simulink model "fft_biplex_test"  (Simulink 7.4)
settings: Solver=VariableStepDiscrete  StartTime=0.0  StopTime=2000  RelTol=1e-3
libraries: xbsIndex_r4 x808, casper_library_misc x46, casper_library_delays x10, casper_library_reorder x2, casper_library_ffts_twiddle x1
(part 3 of 8)

== system fft_biplex_test/fft_biplex/biplex_core/fft_stage_7 ==
  in1 : Inport  OutDataType=sfix(16)  OutScaling=2^0
  in2 : Inport  Port=2  OutDataType=sfix(16)  OutScaling=2^0
  of_in : Inport  Port=3  OutDataType=sfix(16)  OutScaling=2^0
  sync : Inport  Port=4  OutDataType=sfix(16)  OutScaling=2^0
  shift : Inport  Port=5  OutDataType=sfix(16)  OutScaling=2^0
  Counter : xbsIndex_r4/Counter  cnt_type=Free Running  cnt_to=Inf  operation=Up  start_count=0  cnt_by_val=1  arith_type=Unsigned  n_bits=FFTSize-FFTStage+1  bin_pt=0  load_pin=off  rst=on  en=off  explicit_period=off  period=1  dbl_ovrd=off  use_behavioral_HDL=off  implementation=Fabric  use_rpm=off  block_type=counter
      settings: xl_area=[0, 0, 0, 0, 0, 0, 0]  block_version=9.1.01
  Delay : xbsIndex_r4/Delay  en=off  latency=1  dbl_ovrd=off  reg_retiming=off  block_type=delay
      settings: xl_area=[0, 0, 0, 0, 0, 0, 0]  block_version=9.1.01
  Logical1 : xbsIndex_r4/Logical  logical_function=OR  inputs=2  en=off  latency=1  precision=Full  arith_type=Unsigned  n_bits=8  bin_pt=2  align_bp=on  dbl_ovrd=off  block_type=logical
      settings: xl_area=[0, 0, 0, 0, 0, 0, 0]  block_version=9.1.01
  Mux : xbsIndex_r4/Mux  inputs=2  en=off  latency=1  precision=Full  arith_type="Signed  (2's comp)"  n_bits=8  bin_pt=2  quantization=Truncate  overflow=Wrap  dbl_ovrd=off  block_type=mux
      settings: xl_area=[0, 0, 0, 0, 0, 0, 0]  block_version=9.1.01
  Mux1 : xbsIndex_r4/Mux  inputs=2  en=off  latency=1  precision=Full  arith_type="Signed  (2's comp)"  n_bits=8  bin_pt=2  quantization=Truncate  overflow=Wrap  dbl_ovrd=off  block_type=mux
      settings: xl_area=[0, 0, 0, 0, 0, 0, 0]  block_version=9.1.01
  Slice : xbsIndex_r4/Slice  nbits=1  boolean_output=on  mode=Lower Bit Location + Width  bit1=-(FFTStage - 1)  base1=MSB of Input  bit0=FFTStage - 1  base0=LSB of Input  dbl_ovrd=off  block_type=slice
      settings: infoedit="Extracts a given range of bits from each input sample and presents it at the output.  The output type is ordinarily unsigned with binary point at zero, but can be Boolean when the slice is one bit wide.<P><P>Hardware notes: In hardware this block costs nothing."  block_version=9.1.01
  Slice1 : xbsIndex_r4/Slice  nbits=1  boolean_output=off  mode=Upper Bit Location + Width  bit1=0  base1=MSB of Input  bit0=0  base0=LSB of Input  dbl_ovrd=off  block_type=slice
      settings: infoedit="Extracts a given range of bits from each input sample and presents it at the output.  The output type is ordinarily unsigned with binary point at zero, but can be Boolean when the slice is one bit wide.<P><P>Hardware notes: In hardware this block costs nothing."  block_version=9.1.01
  butterfly_direct : Subsystem  AncestorBlock=casper_library_ffts/butterfly_direct  mask(butterfly_direct){biplex=on, FFTSize=8, Coeffs=getfield( getfield( get_param( gcb,'UserData' ), 'parameters'),'Coeffs'), StepPeriod=1, coeff_bit_width=12, input_bit_width=12, downshift=off, add_latency=2, mult_latency=3, bram_latency=2, conv_latency=2, quantization=Round  (unbiased: +/- Inf), overflow=Saturate, arch=Virtex2Pro, opt_target=multipliers, coeffs_bram=on, use_hdl=on, use_embedded=off, hardcode_shifts=off, dsp48_adders=off}
      mask prompts: biplex "Used in biplex FFT"; FFTSize "Size of FFT: (2^? pts)"; Coeffs "Coefficients: (0 to 2^(FFTSize-1)-1)"; StepPeriod "Coefficient Step Period: (2^?)"; coeff_bit_width "Coefficient Bit Width"; input_bit_width "Input/Output Bit Width:"; add_latency "Add Latency"; mult_latency "Mult Latency"; bram_latency "BRAM Latency"; conv_latency "Convert latency"; quantization "Quantization Behavior"; overflow "Overflow Behavior"; arch "Architecture"; opt_target "Use less"; coeffs_bram "Store coefficients in BRAM"; use_hdl "Use behavioural HDL for multipliers"; use_embedded "Use embedded multipliers"; hardcode_shifts "Hardcode shift schedule"; dsp48_adders "Use DSP48s for adders"
      mask help: FFT internal block.
      mask init: same as fft_biplex_test/fft_biplex/biplex_core/fft_stage_1/butterfly_direct
      settings: AttributesFormatString=|
      | twiddle_general_3mult
      | coeffs in BRAM
      mask StyleString: checkbox,edit,edit,edit,edit,edit,checkbox,edit,edit,edit,edit,popup(Truncate|Round  (unbiased: +/- Inf)|Round  (unbiased: Even Values)),popup(Wrap|Saturate|Error),popup(Virtex2Pro|Virtex5),popup(logic|multipliers),checkbox,checkbox,checkbox,checkbox,checkbox
      mask CallbackString:
      | ||Coeffs = get_param(gcb, 'Coeffs');
      | if (length(eval(Coeffs)) == 1),
      |     set_param_state(gcb, 'StepPeriod', 'off');
      |     set_param_state(gcb, 'coeffs_bram', 'off');
      |     set_param_state(gcb, 'coeff_bit_width', 'off');
      | else
      |     set_param_state(gcb, 'StepPeriod', 'on');
      |     set_param_state(gcb, 'coeffs_bram', 'on');
      |     set_param_state(gcb, 'coeff_bit_width', 'on');
      | end|||||||||||fft_callback_arch(gcb);|||% make mutually exclusive with use_embedded.
      | 
      | use_hdl = get_param(gcb, 'use_hdl');
      | if strcmp(use_hdl, 'on'),
      |     set_param_state(gcb, 'use_embedded', 'off');
      | else
      |     set_param_state(gcb, 'use_embedded', 'on');
      | end|% make mutually exclusive with use_hdl.
      | 
      | use_hdl = get_param(gcb, 'use_embedded');
      | if strcmp(use_hdl, 'on'),
      |     set_param_state(gcb, 'use_hdl', 'off');
      | else
      |     set_param_state(gcb, 'use_hdl', 'on');
      | end|hardcode_shifts = get_param(gcb, 'hardcode_shifts');
      | set_param_state(gcb, 'downshift', hardcode_shifts);|fft_callback_dsp48_adders(gcb);
      mask TabNameString: Basic,Basic,Basic,Basic,Basic,Basic,Basic,Latency,Latency,Latency,Latency,Implementation,Implementation,Implementation,Implementation,Implementation,Implementation,Implementation,Implementation,Implementation
  delay_b : Subsystem  AncestorBlock=casper_library_delays/delay_slr  mask(delay_slr){DelayLen=2^(FFTSize-FFTStage)}
      mask prompts: DelayLen "Delay by:"
      mask help: A delay block that uses slices (SLR16s) for its storage.
      mask Help: eval('xlWeb(''http://casper.berkeley.edu/wiki/Delay_slr'')')
  delay_f : Subsystem  AncestorBlock=casper_library_delays/delay_slr  mask(delay_slr){DelayLen=2^(FFTSize-FFTStage)}
      mask prompts: DelayLen "Delay by:"
      mask help: A delay block that uses slices (SLR16s) for its storage.
      mask Help: eval('xlWeb(''http://casper.berkeley.edu/wiki/Delay_slr'')')
  sync_delay : casper_library_delays/sync_delay  SystemSampleTime=-1  DelayLen=2^(FFTSize - FFTStage)
  out1 : Outport  OutDataType=sfix(16)  OutScaling=2^0
  out2 : Outport  Port=2  OutDataType=sfix(16)  OutScaling=2^0
  of : Outport  Port=3  OutDataType=sfix(16)  OutScaling=2^0
  sync_out : Outport  Port=4  OutDataType=sfix(16)  OutScaling=2^0
  wires:
  shift/1 -> Slice/1
  of_in/1 -> Logical1/2
  Logical1/1 -> of/1
  Delay/1 -> sync_delay/1
  sync/1 -> Counter/1, Delay/1
  Counter/1 -> Slice1/1
  Mux/1 -> butterfly_direct/2(b)
  Mux1/1 -> delay_b/1(In1)
  delay_f/1(Out1) -> Mux1/3, Mux/2
  in1/1 -> Mux/3, Mux1/2
  Slice1/1 -> Mux/1, Mux1/1
  in2/1 -> delay_f/1(In1)
  delay_b/1(Out1) -> butterfly_direct/1(a)
  sync_delay/1 -> butterfly_direct/3(sync)
  Slice/1 -> butterfly_direct/4(shift)
  butterfly_direct/1(a+bw) -> out1/1
  butterfly_direct/2(a-bw) -> out2/1
  butterfly_direct/3(of) -> Logical1/1
  butterfly_direct/4(sync_out) -> sync_out/1

== system fft_biplex_test/fft_biplex/biplex_core/fft_stage_8 ==
  in1 : Inport  OutDataType=sfix(16)  OutScaling=2^0
  in2 : Inport  Port=2  OutDataType=sfix(16)  OutScaling=2^0
  of_in : Inport  Port=3  OutDataType=sfix(16)  OutScaling=2^0
  sync : Inport  Port=4  OutDataType=sfix(16)  OutScaling=2^0
  shift : Inport  Port=5  OutDataType=sfix(16)  OutScaling=2^0
  Counter : xbsIndex_r4/Counter  cnt_type=Free Running  cnt_to=Inf  operation=Up  start_count=0  cnt_by_val=1  arith_type=Unsigned  n_bits=FFTSize-FFTStage+1  bin_pt=0  load_pin=off  rst=on  en=off  explicit_period=off  period=1  dbl_ovrd=off  use_behavioral_HDL=off  implementation=Fabric  use_rpm=off  block_type=counter
      settings: xl_area=[0, 0, 0, 0, 0, 0, 0]  block_version=9.1.01
  Delay : xbsIndex_r4/Delay  en=off  latency=1  dbl_ovrd=off  reg_retiming=off  block_type=delay
      settings: xl_area=[0, 0, 0, 0, 0, 0, 0]  block_version=9.1.01
  Logical1 : xbsIndex_r4/Logical  logical_function=OR  inputs=2  en=off  latency=1  precision=Full  arith_type=Unsigned  n_bits=8  bin_pt=2  align_bp=on  dbl_ovrd=off  block_type=logical
      settings: xl_area=[0, 0, 0, 0, 0, 0, 0]  block_version=9.1.01
  Mux : xbsIndex_r4/Mux  inputs=2  en=off  latency=1  precision=Full  arith_type="Signed  (2's comp)"  n_bits=8  bin_pt=2  quantization=Truncate  overflow=Wrap  dbl_ovrd=off  block_type=mux
      settings: xl_area=[0, 0, 0, 0, 0, 0, 0]  block_version=9.1.01
  Mux1 : xbsIndex_r4/Mux  inputs=2  en=off  latency=1  precision=Full  arith_type="Signed  (2's comp)"  n_bits=8  bin_pt=2  quantization=Truncate  overflow=Wrap  dbl_ovrd=off  block_type=mux
      settings: xl_area=[0, 0, 0, 0, 0, 0, 0]  block_version=9.1.01
  Slice : xbsIndex_r4/Slice  nbits=1  boolean_output=on  mode=Lower Bit Location + Width  bit1=-(FFTStage - 1)  base1=MSB of Input  bit0=FFTStage - 1  base0=LSB of Input  dbl_ovrd=off  block_type=slice
      settings: infoedit="Extracts a given range of bits from each input sample and presents it at the output.  The output type is ordinarily unsigned with binary point at zero, but can be Boolean when the slice is one bit wide.<P><P>Hardware notes: In hardware this block costs nothing."  block_version=9.1.01
  Slice1 : xbsIndex_r4/Slice  nbits=1  boolean_output=off  mode=Upper Bit Location + Width  bit1=0  base1=MSB of Input  bit0=0  base0=LSB of Input  dbl_ovrd=off  block_type=slice
      settings: infoedit="Extracts a given range of bits from each input sample and presents it at the output.  The output type is ordinarily unsigned with binary point at zero, but can be Boolean when the slice is one bit wide.<P><P>Hardware notes: In hardware this block costs nothing."  block_version=9.1.01
  butterfly_direct : Subsystem  AncestorBlock=casper_library_ffts/butterfly_direct  mask(butterfly_direct){biplex=on, FFTSize=8, Coeffs=getfield( getfield( get_param( gcb,'UserData' ), 'parameters'),'Coeffs'), StepPeriod=0, coeff_bit_width=12, input_bit_width=12, downshift=off, add_latency=2, mult_latency=3, bram_latency=2, conv_latency=2, quantization=Round  (unbiased: +/- Inf), overflow=Saturate, arch=Virtex2Pro, opt_target=multipliers, coeffs_bram=on, use_hdl=on, use_embedded=off, hardcode_shifts=off, dsp48_adders=off}
      mask prompts: biplex "Used in biplex FFT"; FFTSize "Size of FFT: (2^? pts)"; Coeffs "Coefficients: (0 to 2^(FFTSize-1)-1)"; StepPeriod "Coefficient Step Period: (2^?)"; coeff_bit_width "Coefficient Bit Width"; input_bit_width "Input/Output Bit Width:"; add_latency "Add Latency"; mult_latency "Mult Latency"; bram_latency "BRAM Latency"; conv_latency "Convert latency"; quantization "Quantization Behavior"; overflow "Overflow Behavior"; arch "Architecture"; opt_target "Use less"; coeffs_bram "Store coefficients in BRAM"; use_hdl "Use behavioural HDL for multipliers"; use_embedded "Use embedded multipliers"; hardcode_shifts "Hardcode shift schedule"; dsp48_adders "Use DSP48s for adders"
      mask help: FFT internal block.
      mask init: same as fft_biplex_test/fft_biplex/biplex_core/fft_stage_1/butterfly_direct
      settings: AttributesFormatString=|
      | twiddle_general_3mult
      | coeffs in BRAM
      mask StyleString: checkbox,edit,edit,edit,edit,edit,checkbox,edit,edit,edit,edit,popup(Truncate|Round  (unbiased: +/- Inf)|Round  (unbiased: Even Values)),popup(Wrap|Saturate|Error),popup(Virtex2Pro|Virtex5),popup(logic|multipliers),checkbox,checkbox,checkbox,checkbox,checkbox
      mask CallbackString:
      | ||Coeffs = get_param(gcb, 'Coeffs');
      | if (length(eval(Coeffs)) == 1),
      |     set_param_state(gcb, 'StepPeriod', 'off');
      |     set_param_state(gcb, 'coeffs_bram', 'off');
      |     set_param_state(gcb, 'coeff_bit_width', 'off');
      | else
      |     set_param_state(gcb, 'StepPeriod', 'on');
      |     set_param_state(gcb, 'coeffs_bram', 'on');
      |     set_param_state(gcb, 'coeff_bit_width', 'on');
      | end|||||||||||fft_callback_arch(gcb);|||% make mutually exclusive with use_embedded.
      | 
      | use_hdl = get_param(gcb, 'use_hdl');
      | if strcmp(use_hdl, 'on'),
      |     set_param_state(gcb, 'use_embedded', 'off');
      | else
      |     set_param_state(gcb, 'use_embedded', 'on');
      | end|% make mutually exclusive with use_hdl.
      | 
      | use_hdl = get_param(gcb, 'use_embedded');
      | if strcmp(use_hdl, 'on'),
      |     set_param_state(gcb, 'use_hdl', 'off');
      | else
      |     set_param_state(gcb, 'use_hdl', 'on');
      | end|hardcode_shifts = get_param(gcb, 'hardcode_shifts');
      | set_param_state(gcb, 'downshift', hardcode_shifts);|fft_callback_dsp48_adders(gcb);
      mask TabNameString: Basic,Basic,Basic,Basic,Basic,Basic,Basic,Latency,Latency,Latency,Latency,Implementation,Implementation,Implementation,Implementation,Implementation,Implementation,Implementation,Implementation,Implementation
  delay_b : Subsystem  AncestorBlock=casper_library_delays/delay_slr  mask(delay_slr){DelayLen=2^(FFTSize-FFTStage)}
      mask prompts: DelayLen "Delay by:"
      mask help: A delay block that uses slices (SLR16s) for its storage.
      mask Help: eval('xlWeb(''http://casper.berkeley.edu/wiki/Delay_slr'')')
  delay_f : Subsystem  AncestorBlock=casper_library_delays/delay_slr  mask(delay_slr){DelayLen=2^(FFTSize-FFTStage)}
      mask prompts: DelayLen "Delay by:"
      mask help: A delay block that uses slices (SLR16s) for its storage.
      mask Help: eval('xlWeb(''http://casper.berkeley.edu/wiki/Delay_slr'')')
  sync_delay : casper_library_delays/sync_delay  SystemSampleTime=-1  DelayLen=2^(FFTSize - FFTStage)
  out1 : Outport  OutDataType=sfix(16)  OutScaling=2^0
  out2 : Outport  Port=2  OutDataType=sfix(16)  OutScaling=2^0
  of : Outport  Port=3  OutDataType=sfix(16)  OutScaling=2^0
  sync_out : Outport  Port=4  OutDataType=sfix(16)  OutScaling=2^0
  wires:
  shift/1 -> Slice/1
  of_in/1 -> Logical1/2
  Logical1/1 -> of/1
  Delay/1 -> sync_delay/1
  sync/1 -> Counter/1, Delay/1
  Counter/1 -> Slice1/1
  Mux/1 -> butterfly_direct/2(b)
  Mux1/1 -> delay_b/1(In1)
  delay_f/1(Out1) -> Mux1/3, Mux/2
  in1/1 -> Mux/3, Mux1/2
  Slice1/1 -> Mux/1, Mux1/1
  in2/1 -> delay_f/1(In1)
  delay_b/1(Out1) -> butterfly_direct/1(a)
  sync_delay/1 -> butterfly_direct/3(sync)
  Slice/1 -> butterfly_direct/4(shift)
  butterfly_direct/1(a+bw) -> out1/1
  butterfly_direct/2(a-bw) -> out2/1
  butterfly_direct/3(of) -> Logical1/1
  butterfly_direct/4(sync_out) -> sync_out/1

== system fft_biplex_test/fft_biplex/biplex_cplx_unscrambler/reorder ==
  sync : Inport  OutDataType=sfix(16)  OutScaling=2^0
  en : Inport  Port=2  OutDataType=sfix(16)  OutScaling=2^0
  din0 : Inport  Port=3  OutDataType=sfix(16)  OutScaling=2^0
  Counter : xbsIndex_r4/Counter  cnt_type=Count Limited  cnt_to=511  operation=Up  start_count=0  cnt_by_val=1  arith_type=Unsigned  n_bits=9  bin_pt=0  load_pin=off  rst=on  en=on  explicit_period=on  period=1  dbl_ovrd=off  use_behavioral_HDL=off  implementation=Fabric  block_type=counter
      settings: block_version=11.4
  Mux : xbsIndex_r4/Mux  inputs=2  en=off  latency=1  precision=Full  arith_type=Unsigned  n_bits=16  bin_pt=14  quantization=Truncate  overflow=Wrap  dbl_ovrd=off  block_type=mux
      settings: block_version=11.4
  Slice1 : xbsIndex_r4/Slice  nbits=1  boolean_output=off  mode=Upper Bit Location + Width  bit1=0  base1=MSB of Input  bit0=0  base0=LSB of Input  dbl_ovrd=off  block_type=slice
  Slice2 : xbsIndex_r4/Slice  nbits=8  boolean_output=off  mode=Lower Bit Location + Width  bit1=0  base1=MSB of Input  bit0=0  base0=LSB of Input  dbl_ovrd=off  block_type=slice
  bram0 : xbsIndex_r4/Single Port RAM  depth=256  initVector=sin(pi*(0:15)/16)  distributed_mem=Block RAM  write_mode=Read Before Write  rst=off  init_reg=0  en=off  latency=2  dbl_ovrd=off  optimize=Area  use_rpm=on  block_type=spram
  delay_d0 : xbsIndex_r4/Delay  en=off  latency=0  dbl_ovrd=off  reg_retiming=off  block_type=delay
      settings: block_version=11.4
  delay_din0 : xbsIndex_r4/Delay  en=off  latency=1  dbl_ovrd=off  reg_retiming=off  block_type=delay
      settings: xl_area=[0, 0, 0, 0, 0, 0, 0]  block_version=9.1.01
  delay_map1 : xbsIndex_r4/Delay  en=off  latency=0*map_latency  dbl_ovrd=off  reg_retiming=off  block_type=delay
      settings: block_version=11.4
  delay_sel : xbsIndex_r4/Delay  en=off  latency=0  dbl_ovrd=off  reg_retiming=off  block_type=delay
      settings: block_version=11.4
  delay_valid : xbsIndex_r4/Delay  en=off  latency=3  dbl_ovrd=off  reg_retiming=off  block_type=delay
      settings: xl_area=[0, 0, 0, 0, 0, 0, 0]  block_version=9.1.01
  delay_we : xbsIndex_r4/Delay  en=off  latency=0  dbl_ovrd=off  reg_retiming=off  block_type=delay
      settings: xl_area=[0, 0, 0, 0, 0, 0, 0]  block_version=9.1.01
  map1 : xbsIndex_r4/ROM  depth=256  initVector=map  distributed_mem=Distributed memory  rst=off  init_reg=0  en=off  latency=0  arith_type=Unsigned  n_bits=8  bin_pt=0  dbl_ovrd=off  optimize=Area  use_rpm=on  block_type=sprom
      settings: block_version=11.4
  post_sync_delay : xbsIndex_r4/Delay  en=off  latency=3  dbl_ovrd=off  reg_retiming=off  block_type=delay
      settings: xl_area=[0, 0, 0, 0, 0, 0, 0]  block_version=9.1.01
  pre_sync_delay : xbsIndex_r4/Delay  en=off  latency=0  dbl_ovrd=off  reg_retiming=off  block_type=delay
      settings: xl_area=[0, 0, 0, 0, 0, 0, 0]  block_version=9.1.01
  sync_delay_en : casper_library_delays/sync_delay_en  SystemSampleTime=-1  DelayLen=256
  sync_out : Outport  OutDataType=sfix(16)  OutScaling=2^0
  valid : Outport  Port=2  OutDataType=sfix(16)  OutScaling=2^0
  dout0 : Outport  Port=3  OutDataType=sfix(16)  OutScaling=2^0
  wires:
  sync/1 -> Counter/1, pre_sync_delay/1
  en/1 -> Counter/2, sync_delay_en/2, delay_we/1
  Counter/1 -> Slice1/1, Slice2/1
  Slice1/1 -> delay_sel/1
  delay_sel/1 -> Mux/1
  Slice2/1 -> delay_d0/1, map1/1
  delay_d0/1 -> Mux/2
  pre_sync_delay/1 -> sync_delay_en/1
  sync_delay_en/1 -> post_sync_delay/1
  post_sync_delay/1 -> sync_out/1
  delay_we/1 -> delay_valid/1, bram0/3
  delay_valid/1 -> valid/1
  Mux/1 -> bram0/1
  din0/1 -> delay_din0/1
  delay_din0/1 -> bram0/2
  bram0/1 -> dout0/1
  map1/1 -> delay_map1/1
  delay_map1/1 -> Mux/3

== system fft_biplex_test/fft_biplex/biplex_cplx_unscrambler/reorder1 ==
  sync : Inport  OutDataType=sfix(16)  OutScaling=2^0
  en : Inport  Port=2  OutDataType=sfix(16)  OutScaling=2^0
  din0 : Inport  Port=3  OutDataType=sfix(16)  OutScaling=2^0
  Counter : xbsIndex_r4/Counter  cnt_type=Count Limited  cnt_to=511  operation=Up  start_count=0  cnt_by_val=1  arith_type=Unsigned  n_bits=9  bin_pt=0  load_pin=off  rst=on  en=on  explicit_period=on  period=1  dbl_ovrd=off  use_behavioral_HDL=off  implementation=Fabric  block_type=counter
      settings: block_version=11.4
  Mux : xbsIndex_r4/Mux  inputs=2  en=off  latency=1  precision=Full  arith_type=Unsigned  n_bits=16  bin_pt=14  quantization=Truncate  overflow=Wrap  dbl_ovrd=off  block_type=mux
      settings: block_version=11.4
  Slice1 : xbsIndex_r4/Slice  nbits=1  boolean_output=off  mode=Upper Bit Location + Width  bit1=0  base1=MSB of Input  bit0=0  base0=LSB of Input  dbl_ovrd=off  block_type=slice
  Slice2 : xbsIndex_r4/Slice  nbits=8  boolean_output=off  mode=Lower Bit Location + Width  bit1=0  base1=MSB of Input  bit0=0  base0=LSB of Input  dbl_ovrd=off  block_type=slice
  bram0 : xbsIndex_r4/Single Port RAM  depth=256  initVector=sin(pi*(0:15)/16)  distributed_mem=Block RAM  write_mode=Read Before Write  rst=off  init_reg=0  en=off  latency=2  dbl_ovrd=off  optimize=Area  use_rpm=on  block_type=spram
  delay_d0 : xbsIndex_r4/Delay  en=off  latency=0  dbl_ovrd=off  reg_retiming=off  block_type=delay
      settings: block_version=11.4
  delay_din0 : xbsIndex_r4/Delay  en=off  latency=1  dbl_ovrd=off  reg_retiming=off  block_type=delay
      settings: xl_area=[0, 0, 0, 0, 0, 0, 0]  block_version=9.1.01
  delay_map1 : xbsIndex_r4/Delay  en=off  latency=0*map_latency  dbl_ovrd=off  reg_retiming=off  block_type=delay
      settings: block_version=11.4
  delay_sel : xbsIndex_r4/Delay  en=off  latency=0  dbl_ovrd=off  reg_retiming=off  block_type=delay
      settings: block_version=11.4
  delay_valid : xbsIndex_r4/Delay  en=off  latency=3  dbl_ovrd=off  reg_retiming=off  block_type=delay
      settings: xl_area=[0, 0, 0, 0, 0, 0, 0]  block_version=9.1.01
  delay_we : xbsIndex_r4/Delay  en=off  latency=0  dbl_ovrd=off  reg_retiming=off  block_type=delay
      settings: xl_area=[0, 0, 0, 0, 0, 0, 0]  block_version=9.1.01
  map1 : xbsIndex_r4/ROM  depth=256  initVector=map  distributed_mem=Distributed memory  rst=off  init_reg=0  en=off  latency=0  arith_type=Unsigned  n_bits=8  bin_pt=0  dbl_ovrd=off  optimize=Area  use_rpm=on  block_type=sprom
      settings: block_version=11.4
  post_sync_delay : xbsIndex_r4/Delay  en=off  latency=3  dbl_ovrd=off  reg_retiming=off  block_type=delay
      settings: xl_area=[0, 0, 0, 0, 0, 0, 0]  block_version=9.1.01
  pre_sync_delay : xbsIndex_r4/Delay  en=off  latency=0  dbl_ovrd=off  reg_retiming=off  block_type=delay
      settings: xl_area=[0, 0, 0, 0, 0, 0, 0]  block_version=9.1.01
  sync_delay_en : casper_library_delays/sync_delay_en  SystemSampleTime=-1  DelayLen=256
  sync_out : Outport  OutDataType=sfix(16)  OutScaling=2^0
  valid : Outport  Port=2  OutDataType=sfix(16)  OutScaling=2^0
  dout0 : Outport  Port=3  OutDataType=sfix(16)  OutScaling=2^0
  wires:
  sync/1 -> Counter/1, pre_sync_delay/1
  en/1 -> Counter/2, sync_delay_en/2, delay_we/1
  Counter/1 -> Slice1/1, Slice2/1
  Slice1/1 -> delay_sel/1
  delay_sel/1 -> Mux/1
  Slice2/1 -> delay_d0/1, map1/1
  delay_d0/1 -> Mux/2
  pre_sync_delay/1 -> sync_delay_en/1
  sync_delay_en/1 -> post_sync_delay/1
  post_sync_delay/1 -> sync_out/1
  delay_we/1 -> delay_valid/1, bram0/3
  delay_valid/1 -> valid/1
  Mux/1 -> bram0/1
  din0/1 -> delay_din0/1
  delay_din0/1 -> bram0/2
  bram0/1 -> dout0/1
  map1/1 -> delay_map1/1
  delay_map1/1 -> Mux/3

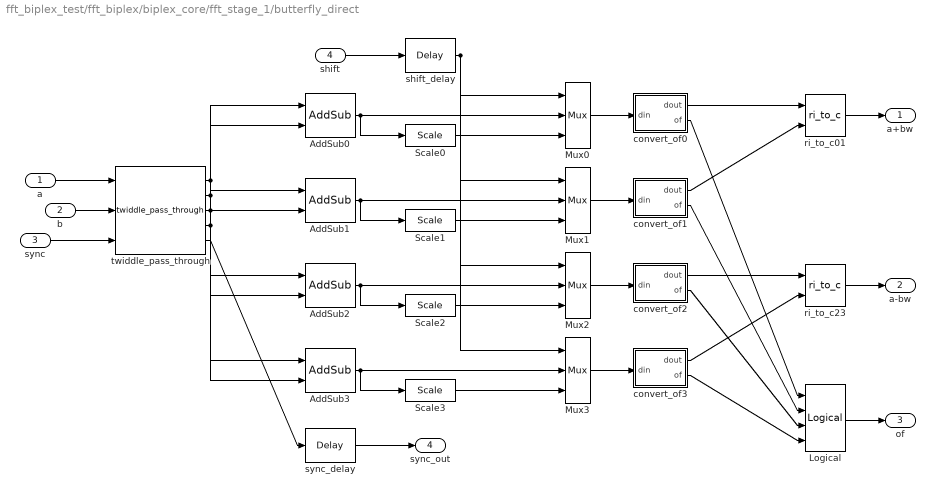
== system fft_biplex_test/fft_biplex/biplex_core/fft_stage_1/butterfly_direct ==
  a : Inport  OutDataType=sfix(16)  OutScaling=2^0
  b : Inport  Port=2  OutDataType=sfix(16)  OutScaling=2^0
  sync : Inport  Port=3  OutDataType=sfix(16)  OutScaling=2^0
  shift : Inport  Port=4  OutDataType=sfix(16)  OutScaling=2^0
  AddSub0 : xbsIndex_r4/AddSub  mode=Addition  use_carryin=off  use_carryout=off  en=off  latency=2  precision=Full  arith_type=Unsigned  n_bits=16  bin_pt=14  quantization=Truncate  overflow=Wrap  dbl_ovrd=off  use_behavioral_HDL=on  hw_selection=Fabric  pipelined=off  block_type=addsub
  AddSub1 : xbsIndex_r4/AddSub  mode=Addition  use_carryin=off  use_carryout=off  en=off  latency=2  precision=Full  arith_type=Unsigned  n_bits=16  bin_pt=14  quantization=Truncate  overflow=Wrap  dbl_ovrd=off  use_behavioral_HDL=on  hw_selection=Fabric  pipelined=off  block_type=addsub
  AddSub2 : xbsIndex_r4/AddSub  mode=Subtraction  use_carryin=off  use_carryout=off  en=off  latency=2  precision=Full  arith_type=Unsigned  n_bits=16  bin_pt=14  quantization=Truncate  overflow=Wrap  dbl_ovrd=off  use_behavioral_HDL=on  hw_selection=Fabric  pipelined=off  block_type=addsub
  AddSub3 : xbsIndex_r4/AddSub  mode=Subtraction  use_carryin=off  use_carryout=off  en=off  latency=2  precision=Full  arith_type=Unsigned  n_bits=16  bin_pt=14  quantization=Truncate  overflow=Wrap  dbl_ovrd=off  use_behavioral_HDL=on  hw_selection=Fabric  pipelined=off  block_type=addsub
  Logical : xbsIndex_r4/Logical  logical_function=OR  inputs=4  en=off  latency=0  precision=Full  arith_type=Unsigned  n_bits=16  bin_pt=0  align_bp=on  dbl_ovrd=off  block_type=logical
      settings: block_version=11.4
  Mux{0..3} (4 alike) : xbsIndex_r4/Mux  inputs=2  en=off  latency=1  precision=Full  arith_type=Unsigned  n_bits=16  bin_pt=14  quantization=Truncate  overflow=Wrap  dbl_ovrd=off  block_type=mux
      settings: block_version=11.4
  Scale{0..3} (4 alike) : xbsIndex_r4/Scale  scale_factor=-1  dbl_ovrd=off  block_type=scale
  convert_of0 : Subsystem  AncestorBlock=casper_library_misc/convert_of  mask(convert_of){bit_width_i=14, binary_point_i=12, bit_width_o=12, binary_point_o=11, latency=2, overflow=Saturate, quantization=Round  (unbiased: +/- Inf)}
      mask prompts: bit_width_i "Bit Width In"; binary_point_i "Binary Point In"; bit_width_o "Bit Width Out"; binary_point_o "Binary Point Out"; overflow "Overflow Behaviour"; quantization "Quantization Behaviour"
      mask help:
      | Converts from one 2's complement bit-width
      | and/or binary point position to another.
      | Includes underflow/overflow indicator.
      mask init:
      | convert_of_init(gcb, ...
      |     'bit_width_i', bit_width_i, ...
      |     'binary_point_i', binary_point_i, ...
      |     'bit_width_o', bit_width_o, ...
      |     'binary_point_o', binary_point_o, ...
      |     'latency', latency, ...
      |     'overflow', overflow, ...
      |     'quantization', quantization);
      settings: AttributesFormatString=[14,12]->[12,11]
      mask StyleString: edit,edit,edit,edit,edit,popup(Wrap|Saturate|Error),popup(Truncate|Round  (unbiased: +/- Inf)|Round  (unbiased: even values))
  convert_of1 : Subsystem  AncestorBlock=casper_library_misc/convert_of  mask(convert_of){bit_width_i=14, binary_point_i=12, bit_width_o=12, binary_point_o=11, latency=2, overflow=Saturate, quantization=Round  (unbiased: +/- Inf)}
      mask prompts: bit_width_i "Bit Width In"; binary_point_i "Binary Point In"; bit_width_o "Bit Width Out"; binary_point_o "Binary Point Out"; overflow "Overflow Behaviour"; quantization "Quantization Behaviour"
      mask help:
      | Converts from one 2's complement bit-width
      | and/or binary point position to another.
      | Includes underflow/overflow indicator.
      mask init: same as fft_biplex_test/fft_biplex/biplex_core/fft_stage_1/butterfly_direct/convert_of0
      settings: AttributesFormatString=[14,12]->[12,11]
      mask StyleString: edit,edit,edit,edit,edit,popup(Wrap|Saturate|Error),popup(Truncate|Round  (unbiased: +/- Inf)|Round  (unbiased: even values))
  convert_of2 : Subsystem  AncestorBlock=casper_library_misc/convert_of  mask(convert_of){bit_width_i=14, binary_point_i=12, bit_width_o=12, binary_point_o=11, latency=2, overflow=Saturate, quantization=Round  (unbiased: +/- Inf)}
      mask prompts: bit_width_i "Bit Width In"; binary_point_i "Binary Point In"; bit_width_o "Bit Width Out"; binary_point_o "Binary Point Out"; overflow "Overflow Behaviour"; quantization "Quantization Behaviour"
      mask help:
      | Converts from one 2's complement bit-width
      | and/or binary point position to another.
      | Includes underflow/overflow indicator.
      mask init: same as fft_biplex_test/fft_biplex/biplex_core/fft_stage_1/butterfly_direct/convert_of0
      settings: AttributesFormatString=[14,12]->[12,11]
      mask StyleString: edit,edit,edit,edit,edit,popup(Wrap|Saturate|Error),popup(Truncate|Round  (unbiased: +/- Inf)|Round  (unbiased: even values))
  convert_of3 : Subsystem  AncestorBlock=casper_library_misc/convert_of  mask(convert_of){bit_width_i=14, binary_point_i=12, bit_width_o=12, binary_point_o=11, latency=2, overflow=Saturate, quantization=Round  (unbiased: +/- Inf)}
      mask prompts: bit_width_i "Bit Width In"; binary_point_i "Binary Point In"; bit_width_o "Bit Width Out"; binary_point_o "Binary Point Out"; overflow "Overflow Behaviour"; quantization "Quantization Behaviour"
      mask help:
      | Converts from one 2's complement bit-width
      | and/or binary point position to another.
      | Includes underflow/overflow indicator.
      mask init: same as fft_biplex_test/fft_biplex/biplex_core/fft_stage_1/butterfly_direct/convert_of0
      settings: AttributesFormatString=[14,12]->[12,11]
      mask StyleString: edit,edit,edit,edit,edit,popup(Wrap|Saturate|Error),popup(Truncate|Round  (unbiased: +/- Inf)|Round  (unbiased: even values))
  ri_to_c01 : casper_library_misc/ri_to_c  SystemSampleTime=-1
  ri_to_c23 : casper_library_misc/ri_to_c  SystemSampleTime=-1
  shift_delay : xbsIndex_r4/Delay  en=off  latency=2  dbl_ovrd=off  reg_retiming=off  block_type=delay
      settings: block_version=11.4
  sync_delay : xbsIndex_r4/Delay  en=off  latency=5  dbl_ovrd=off  reg_retiming=on  block_type=delay
      settings: block_version=11.4
  twiddle_pass_through : casper_library_ffts_twiddle/twiddle_pass_through  SystemSampleTime=-1  FFTSize=8  input_bit_width=12  add_latency=2  mult_latency=3  bram_latency=2  conv_latency=2  opt_target=multipliers
  a+bw : Outport  OutDataType=sfix(16)  OutScaling=2^0
  a-bw : Outport  Port=2  OutDataType=sfix(16)  OutScaling=2^0
  of : Outport  Port=3  OutDataType=sfix(16)  OutScaling=2^0
  sync_out : Outport  Port=4
  wires:
  a/1 -> twiddle_pass_through/1
  b/1 -> twiddle_pass_through/2
  sync/1 -> twiddle_pass_through/3
  twiddle_pass_through/1 -> AddSub0/1, AddSub2/1
  twiddle_pass_through/2 -> AddSub1/1, AddSub3/1
  twiddle_pass_through/3 -> AddSub0/2, AddSub2/2
  twiddle_pass_through/4 -> AddSub1/2, AddSub3/2
  twiddle_pass_through/5 -> sync_delay/1
  shift/1 -> shift_delay/1
  shift_delay/1 -> Mux0/1, Mux1/1, Mux2/1, Mux3/1
  AddSub0/1 -> Mux0/2, Scale0/1
  AddSub1/1 -> Mux1/2, Scale1/1
  AddSub2/1 -> Mux2/2, Scale2/1
  AddSub3/1 -> Mux3/2, Scale3/1
  Scale0/1 -> Mux0/3
  Scale1/1 -> Mux1/3
  Scale2/1 -> Mux2/3
  Scale3/1 -> Mux3/3
  Mux0/1 -> convert_of0/1(din)
  Mux1/1 -> convert_of1/1(din)
  Mux2/1 -> convert_of2/1(din)
  Mux3/1 -> convert_of3/1(din)
  convert_of0/1(dout) -> ri_to_c01/1
  convert_of1/1(dout) -> ri_to_c01/2
  convert_of2/1(dout) -> ri_to_c23/1
  convert_of3/1(dout) -> ri_to_c23/2
  convert_of0/2(of) -> Logical/1
  convert_of1/2(of) -> Logical/2
  convert_of2/2(of) -> Logical/3
  convert_of3/2(of) -> Logical/4
  ri_to_c01/1 -> a+bw/1
  ri_to_c23/1 -> a-bw/1
  Logical/1 -> of/1
  sync_delay/1 -> sync_out/1

== system fft_biplex_test/fft_biplex/biplex_core/fft_stage_1/delay_b ==
  In1 : Inport  OutDataType=sfix(16)  OutScaling=2^0
  Constant2 : xbsIndex_r4/Constant  arith_type=Boolean  const=1  n_bits=1  bin_pt=0  explicit_period=on  period=1  equ=P=C  opselect=C  inp2=PCIN>>17  opr=+  inp1=P  carry=CIN  dbl_ovrd=off  block_type=constant
      settings: block_version=9.1.01
  Counter : xbsIndex_r4/Counter  cnt_type=Count Limited  cnt_to=DelayLen - bram_latency - 1  operation=Up  start_count=0  cnt_by_val=1  arith_type=Unsigned  n_bits=BitWidth  bin_pt=0  load_pin=off  rst=off  en=off  explicit_period=on  period=1  dbl_ovrd=off  use_behavioral_HDL=off  implementation=Fabric  use_rpm=off  block_type=counter
      settings: xl_area=[0, 0, 0, 0, 0, 0, 0]  block_version=9.1.01
  Single Port RAM : xbsIndex_r4/Single Port RAM  depth=2^BitWidth  initVector=0  distributed_mem=Block RAM  write_mode=Read Before Write  rst=off  init_reg=0  en=off  latency=bram_latency  dbl_ovrd=off  optimize=Area  use_rpm=off  block_type=spram
      settings: xl_area=[0, 0, 0, 0, 0, 0, 0]  block_version=9.1.01
  Out1 : Outport  OutDataType=sfix(16)  OutScaling=2^0
  wires:
  Constant2/1 -> Single Port RAM/3
  In1/1 -> Single Port RAM/2
  Counter/1 -> Single Port RAM/1
  Single Port RAM/1 -> Out1/1

== system fft_biplex_test/fft_biplex/biplex_core/fft_stage_1/delay_f ==
  In1 : Inport  OutDataType=sfix(16)  OutScaling=2^0
  Constant2 : xbsIndex_r4/Constant  arith_type=Boolean  const=1  n_bits=1  bin_pt=0  explicit_period=on  period=1  equ=P=C  opselect=C  inp2=PCIN>>17  opr=+  inp1=P  carry=CIN  dbl_ovrd=off  block_type=constant
      settings: block_version=9.1.01
  Counter : xbsIndex_r4/Counter  cnt_type=Count Limited  cnt_to=DelayLen - bram_latency - 1  operation=Up  start_count=0  cnt_by_val=1  arith_type=Unsigned  n_bits=BitWidth  bin_pt=0  load_pin=off  rst=off  en=off  explicit_period=on  period=1  dbl_ovrd=off  use_behavioral_HDL=off  implementation=Fabric  use_rpm=off  block_type=counter
      settings: xl_area=[0, 0, 0, 0, 0, 0, 0]  block_version=9.1.01
  Single Port RAM : xbsIndex_r4/Single Port RAM  depth=2^BitWidth  initVector=0  distributed_mem=Block RAM  write_mode=Read Before Write  rst=off  init_reg=0  en=off  latency=bram_latency  dbl_ovrd=off  optimize=Area  use_rpm=off  block_type=spram
      settings: xl_area=[0, 0, 0, 0, 0, 0, 0]  block_version=9.1.01
  Out1 : Outport  OutDataType=sfix(16)  OutScaling=2^0
  wires:
  Constant2/1 -> Single Port RAM/3
  In1/1 -> Single Port RAM/2
  Counter/1 -> Single Port RAM/1
  Single Port RAM/1 -> Out1/1

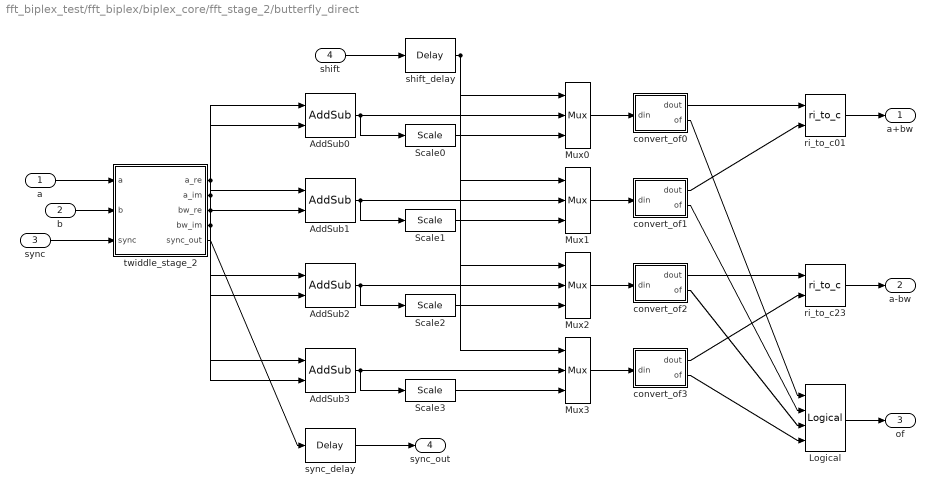
== system fft_biplex_test/fft_biplex/biplex_core/fft_stage_2/butterfly_direct ==
  a : Inport  OutDataType=sfix(16)  OutScaling=2^0
  b : Inport  Port=2  OutDataType=sfix(16)  OutScaling=2^0
  sync : Inport  Port=3  OutDataType=sfix(16)  OutScaling=2^0
  shift : Inport  Port=4  OutDataType=sfix(16)  OutScaling=2^0
  AddSub0 : xbsIndex_r4/AddSub  mode=Addition  use_carryin=off  use_carryout=off  en=off  latency=2  precision=Full  arith_type=Unsigned  n_bits=16  bin_pt=14  quantization=Truncate  overflow=Wrap  dbl_ovrd=off  use_behavioral_HDL=on  hw_selection=Fabric  pipelined=off  block_type=addsub
  AddSub1 : xbsIndex_r4/AddSub  mode=Addition  use_carryin=off  use_carryout=off  en=off  latency=2  precision=Full  arith_type=Unsigned  n_bits=16  bin_pt=14  quantization=Truncate  overflow=Wrap  dbl_ovrd=off  use_behavioral_HDL=on  hw_selection=Fabric  pipelined=off  block_type=addsub
  AddSub2 : xbsIndex_r4/AddSub  mode=Subtraction  use_carryin=off  use_carryout=off  en=off  latency=2  precision=Full  arith_type=Unsigned  n_bits=16  bin_pt=14  quantization=Truncate  overflow=Wrap  dbl_ovrd=off  use_behavioral_HDL=on  hw_selection=Fabric  pipelined=off  block_type=addsub
  AddSub3 : xbsIndex_r4/AddSub  mode=Subtraction  use_carryin=off  use_carryout=off  en=off  latency=2  precision=Full  arith_type=Unsigned  n_bits=16  bin_pt=14  quantization=Truncate  overflow=Wrap  dbl_ovrd=off  use_behavioral_HDL=on  hw_selection=Fabric  pipelined=off  block_type=addsub
  Logical : xbsIndex_r4/Logical  logical_function=OR  inputs=4  en=off  latency=0  precision=Full  arith_type=Unsigned  n_bits=16  bin_pt=0  align_bp=on  dbl_ovrd=off  block_type=logical
      settings: block_version=11.4
  Mux{0..3} (4 alike) : xbsIndex_r4/Mux  inputs=2  en=off  latency=1  precision=Full  arith_type=Unsigned  n_bits=16  bin_pt=14  quantization=Truncate  overflow=Wrap  dbl_ovrd=off  block_type=mux
      settings: block_version=11.4
  Scale{0..3} (4 alike) : xbsIndex_r4/Scale  scale_factor=-1  dbl_ovrd=off  block_type=scale
  convert_of0 : Subsystem  AncestorBlock=casper_library_misc/convert_of  mask(convert_of){bit_width_i=14, binary_point_i=12, bit_width_o=12, binary_point_o=11, latency=2, overflow=Saturate, quantization=Round  (unbiased: +/- Inf)}
      mask prompts: bit_width_i "Bit Width In"; binary_point_i "Binary Point In"; bit_width_o "Bit Width Out"; binary_point_o "Binary Point Out"; overflow "Overflow Behaviour"; quantization "Quantization Behaviour"
      mask help:
      | Converts from one 2's complement bit-width
      | and/or binary point position to another.
      | Includes underflow/overflow indicator.
      mask init: same as fft_biplex_test/fft_biplex/biplex_core/fft_stage_1/butterfly_direct/convert_of0
      settings: AttributesFormatString=[14,12]->[12,11]
      mask StyleString: edit,edit,edit,edit,edit,popup(Wrap|Saturate|Error),popup(Truncate|Round  (unbiased: +/- Inf)|Round  (unbiased: even values))
  convert_of1 : Subsystem  AncestorBlock=casper_library_misc/convert_of  mask(convert_of){bit_width_i=14, binary_point_i=12, bit_width_o=12, binary_point_o=11, latency=2, overflow=Saturate, quantization=Round  (unbiased: +/- Inf)}
      mask prompts: bit_width_i "Bit Width In"; binary_point_i "Binary Point In"; bit_width_o "Bit Width Out"; binary_point_o "Binary Point Out"; overflow "Overflow Behaviour"; quantization "Quantization Behaviour"
      mask help:
      | Converts from one 2's complement bit-width
      | and/or binary point position to another.
      | Includes underflow/overflow indicator.
      mask init: same as fft_biplex_test/fft_biplex/biplex_core/fft_stage_1/butterfly_direct/convert_of0
      settings: AttributesFormatString=[14,12]->[12,11]
      mask StyleString: edit,edit,edit,edit,edit,popup(Wrap|Saturate|Error),popup(Truncate|Round  (unbiased: +/- Inf)|Round  (unbiased: even values))
  convert_of2 : Subsystem  AncestorBlock=casper_library_misc/convert_of  mask(convert_of){bit_width_i=14, binary_point_i=12, bit_width_o=12, binary_point_o=11, latency=2, overflow=Saturate, quantization=Round  (unbiased: +/- Inf)}
      mask prompts: bit_width_i "Bit Width In"; binary_point_i "Binary Point In"; bit_width_o "Bit Width Out"; binary_point_o "Binary Point Out"; overflow "Overflow Behaviour"; quantization "Quantization Behaviour"
      mask help:
      | Converts from one 2's complement bit-width
      | and/or binary point position to another.
      | Includes underflow/overflow indicator.
      mask init: same as fft_biplex_test/fft_biplex/biplex_core/fft_stage_1/butterfly_direct/convert_of0
      settings: AttributesFormatString=[14,12]->[12,11]
      mask StyleString: edit,edit,edit,edit,edit,popup(Wrap|Saturate|Error),popup(Truncate|Round  (unbiased: +/- Inf)|Round  (unbiased: even values))
  convert_of3 : Subsystem  AncestorBlock=casper_library_misc/convert_of  mask(convert_of){bit_width_i=14, binary_point_i=12, bit_width_o=12, binary_point_o=11, latency=2, overflow=Saturate, quantization=Round  (unbiased: +/- Inf)}
      mask prompts: bit_width_i "Bit Width In"; binary_point_i "Binary Point In"; bit_width_o "Bit Width Out"; binary_point_o "Binary Point Out"; overflow "Overflow Behaviour"; quantization "Quantization Behaviour"
      mask help:
      | Converts from one 2's complement bit-width
      | and/or binary point position to another.
      | Includes underflow/overflow indicator.
      mask init: same as fft_biplex_test/fft_biplex/biplex_core/fft_stage_1/butterfly_direct/convert_of0
      settings: AttributesFormatString=[14,12]->[12,11]
      mask StyleString: edit,edit,edit,edit,edit,popup(Wrap|Saturate|Error),popup(Truncate|Round  (unbiased: +/- Inf)|Round  (unbiased: even values))
  ri_to_c01 : casper_library_misc/ri_to_c  SystemSampleTime=-1
  ri_to_c23 : casper_library_misc/ri_to_c  SystemSampleTime=-1
  shift_delay : xbsIndex_r4/Delay  en=off  latency=2  dbl_ovrd=off  reg_retiming=off  block_type=delay
      settings: block_version=11.4
  sync_delay : xbsIndex_r4/Delay  en=off  latency=5  dbl_ovrd=off  reg_retiming=on  block_type=delay
      settings: block_version=11.4
  twiddle_stage_2 : Subsystem  AncestorBlock=casper_library_ffts_twiddle/twiddle_stage_2  mask(twiddle_pass_through){FFTSize=8, input_bit_width=12, add_latency=2, mult_latency=3, bram_latency=2, conv_latency=2, opt_target=multipliers}
      mask prompts: FFTSize "FFT Size (2^?)"; input_bit_width "Input Bit Width"; add_latency "Add Latency"; mult_latency "Mult Latency"; bram_latency "BRAM Latency"; conv_latency "Convert latency"; opt_target "Use less"
      mask help:
      | Used in FFT library. Used when coefficients
      | are 2^0 i.e just pass data through without delays
      mask init:
      | set_param(gcb,'LinkStatus','inactive');
      | if(strcmp(opt_target, 'logic')), 
      |     lat = add_latency;
      |     lat_str = 'add_latency';
      | else,
      |     lat = add_latency*2;
      |     lat_str = 'add_latency*2';
      | end
      | set_param([gcb,'/delay0'], 'latency', ...
      |     ['bram_latency+mult_latency+conv_latency+',lat_str]);
      | set_param([gcb,'/delay1'], 'latency', ...
      |     ['bram_latency+mult_latency+conv_latency+',lat_str]);
      | set_param([gcb,'/mux0'], 'latency', ...
      |     num2str(mult_latency+conv_latency+lat));
      | set_param([gcb,'/mux1'], 'latency', ...
      |     num2str(mult_latency+conv_latency+lat));
      | set_param([gcb,'/delay6'], 'latency', ...
      |     ['mult_latency+conv_latency+',lat_str]);
      mask StyleString: edit,edit,edit,edit,edit,edit,popup(logic|multipliers)
  a+bw : Outport  OutDataType=sfix(16)  OutScaling=2^0
  a-bw : Outport  Port=2  OutDataType=sfix(16)  OutScaling=2^0
  of : Outport  Port=3  OutDataType=sfix(16)  OutScaling=2^0
  sync_out : Outport  Port=4
  wires:
  a/1 -> twiddle_stage_2/1(a)
  b/1 -> twiddle_stage_2/2(b)
  sync/1 -> twiddle_stage_2/3(sync)
  twiddle_stage_2/1(a_re) -> AddSub0/1, AddSub2/1
  twiddle_stage_2/2(a_im) -> AddSub1/1, AddSub3/1
  twiddle_stage_2/3(bw_re) -> AddSub0/2, AddSub2/2
  twiddle_stage_2/4(bw_im) -> AddSub1/2, AddSub3/2
  twiddle_stage_2/5(sync_out) -> sync_delay/1
  shift/1 -> shift_delay/1
  shift_delay/1 -> Mux0/1, Mux1/1, Mux2/1, Mux3/1
  AddSub0/1 -> Mux0/2, Scale0/1
  AddSub1/1 -> Mux1/2, Scale1/1
  AddSub2/1 -> Mux2/2, Scale2/1
  AddSub3/1 -> Mux3/2, Scale3/1
  Scale0/1 -> Mux0/3
  Scale1/1 -> Mux1/3
  Scale2/1 -> Mux2/3
  Scale3/1 -> Mux3/3
  Mux0/1 -> convert_of0/1(din)
  Mux1/1 -> convert_of1/1(din)
  Mux2/1 -> convert_of2/1(din)
  Mux3/1 -> convert_of3/1(din)
  convert_of0/1(dout) -> ri_to_c01/1
  convert_of1/1(dout) -> ri_to_c01/2
  convert_of2/1(dout) -> ri_to_c23/1
  convert_of3/1(dout) -> ri_to_c23/2
  convert_of0/2(of) -> Logical/1
  convert_of1/2(of) -> Logical/2
  convert_of2/2(of) -> Logical/3
  convert_of3/2(of) -> Logical/4
  ri_to_c01/1 -> a+bw/1
  ri_to_c23/1 -> a-bw/1
  Logical/1 -> of/1
  sync_delay/1 -> sync_out/1

== system fft_biplex_test/fft_biplex/biplex_core/fft_stage_2/delay_b ==
  In1 : Inport  OutDataType=sfix(16)  OutScaling=2^0
  Constant2 : xbsIndex_r4/Constant  arith_type=Boolean  const=1  n_bits=1  bin_pt=0  explicit_period=on  period=1  equ=P=C  opselect=C  inp2=PCIN>>17  opr=+  inp1=P  carry=CIN  dbl_ovrd=off  block_type=constant
      settings: block_version=9.1.01
  Counter : xbsIndex_r4/Counter  cnt_type=Count Limited  cnt_to=DelayLen - bram_latency - 1  operation=Up  start_count=0  cnt_by_val=1  arith_type=Unsigned  n_bits=BitWidth  bin_pt=0  load_pin=off  rst=off  en=off  explicit_period=on  period=1  dbl_ovrd=off  use_behavioral_HDL=off  implementation=Fabric  use_rpm=off  block_type=counter
      settings: xl_area=[0, 0, 0, 0, 0, 0, 0]  block_version=9.1.01
  Single Port RAM : xbsIndex_r4/Single Port RAM  depth=2^BitWidth  initVector=0  distributed_mem=Block RAM  write_mode=Read Before Write  rst=off  init_reg=0  en=off  latency=bram_latency  dbl_ovrd=off  optimize=Area  use_rpm=off  block_type=spram
      settings: xl_area=[0, 0, 0, 0, 0, 0, 0]  block_version=9.1.01
  Out1 : Outport  OutDataType=sfix(16)  OutScaling=2^0
  wires:
  Constant2/1 -> Single Port RAM/3
  In1/1 -> Single Port RAM/2
  Counter/1 -> Single Port RAM/1
  Single Port RAM/1 -> Out1/1

== system fft_biplex_test/fft_biplex/biplex_core/fft_stage_2/delay_f ==
  In1 : Inport  OutDataType=sfix(16)  OutScaling=2^0
  Constant2 : xbsIndex_r4/Constant  arith_type=Boolean  const=1  n_bits=1  bin_pt=0  explicit_period=on  period=1  equ=P=C  opselect=C  inp2=PCIN>>17  opr=+  inp1=P  carry=CIN  dbl_ovrd=off  block_type=constant
      settings: block_version=9.1.01
  Counter : xbsIndex_r4/Counter  cnt_type=Count Limited  cnt_to=DelayLen - bram_latency - 1  operation=Up  start_count=0  cnt_by_val=1  arith_type=Unsigned  n_bits=BitWidth  bin_pt=0  load_pin=off  rst=off  en=off  explicit_period=on  period=1  dbl_ovrd=off  use_behavioral_HDL=off  implementation=Fabric  use_rpm=off  block_type=counter
      settings: xl_area=[0, 0, 0, 0, 0, 0, 0]  block_version=9.1.01
  Single Port RAM : xbsIndex_r4/Single Port RAM  depth=2^BitWidth  initVector=0  distributed_mem=Block RAM  write_mode=Read Before Write  rst=off  init_reg=0  en=off  latency=bram_latency  dbl_ovrd=off  optimize=Area  use_rpm=off  block_type=spram
      settings: xl_area=[0, 0, 0, 0, 0, 0, 0]  block_version=9.1.01
  Out1 : Outport  OutDataType=sfix(16)  OutScaling=2^0
  wires:
  Constant2/1 -> Single Port RAM/3
  In1/1 -> Single Port RAM/2
  Counter/1 -> Single Port RAM/1
  Single Port RAM/1 -> Out1/1
